simulink model "TECMD_Prototype"  (R2021a)
settings: Solver=daessc  StartTime=0.0  FixedStep=0.1  RelTol=1e-3  AbsTol=1e-3
libraries: nesl_utility x8, fl_lib x7, BatteryLibrary_lib x2
settings Model: Creator=widana_d  LastModifiedBy=widana_d
settings SolverCC: AutoScaleAbsTol=off  AlgebraicLoopSolver=TrustRegion
settings DataIOCC: SaveState=on
settings DebuggingCC: SymbolicDimsDataTypeCodeGenerationDiagnostic=none  SFMachineParentedDataDiag=warning
settings SFSimCC: CustomCodeUndefinedFunction=UseInterfaceOnly
settings SimscapeCC: SimscapeLogType=all  SimscapeLogSimulationStatistics=on  SimscapeLogDataHistory=10000

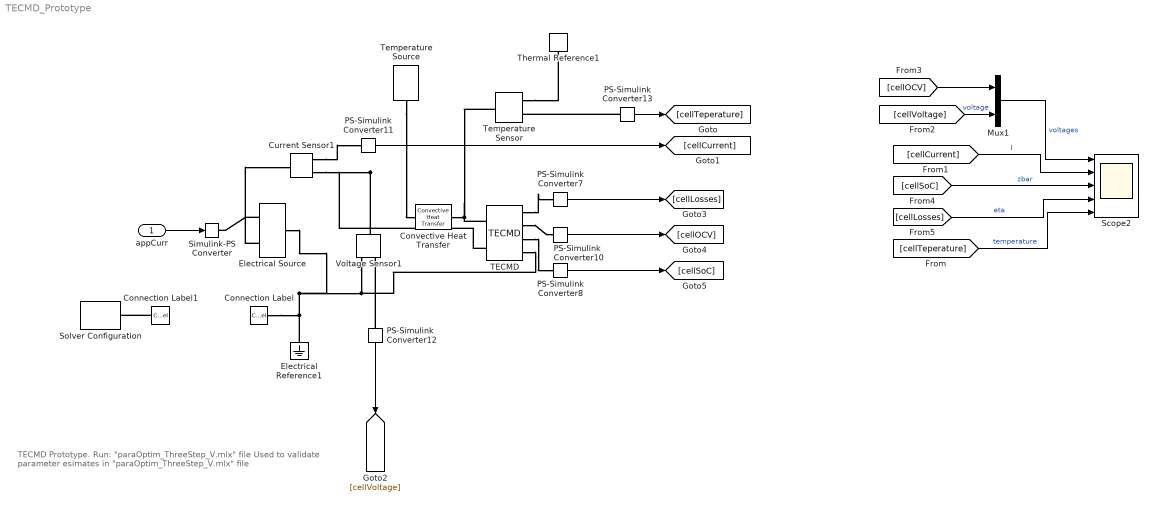
== system TECMD_Prototype ==
  note: TECMD Prototype.
      | Run: "paraOptim_ThreeStep_V.mlx" file
      | Used to validate parameter esimates in "paraOptim_ThreeStep_V.mlx" file
  appCurr : Inport
  Connection Label : ConnectionLabel  Label=solver
  Connection Label1 : ConnectionLabel  Label=solver
  Convective Heat Transfer : fl_lib/Thermal/Thermal Elements/Convective Heat Transfer  area=cellArea m^2  heat_tr_coeff=h W/(m^2 * K)  T_specify=off  T_priority=None  T=0 K  T_nominal_specify=off  T_nominal_unit=K  T_nominal_value=1  Q_specify=off  Q_priority=None  Q=0 W  Q_nominal_specify=off  Q_nominal_unit=W  Q_nominal_value=1
  Current Sensor1 : fl_lib/Electrical/Electrical Sensors/Current Sensor
  Electrical Reference1 : fl_lib/Electrical/Electrical Elements/Electrical Reference
  Electrical Source : BatteryLibrary_lib/Utilities/Electrical Source  inType=0
      settings: InternalSimscapePortConfiguration="{\"Bottom\":[{\"id\":\"n\",\"label\":\"-\",\"type\":\"foundation.electrical.electrical\"}],\"Left\":[{\"id\":\"inputSignal\",\"label\":\"Input\",\"type\":\"input\"}],\"Right\":[],\"Top\":[{\"id\":\"p\",\"label\":\"+\",\"type\":\"foundation.electrical.electrical\"}]}"
  Mux1 : Mux  Inputs=2
  PS-Simulink Converter{7..8,10..13} (6 alike) : nesl_utility/PS-Simulink Converter  PhysicalDomain=network_engine_domain  SubClassName=ps_output  LeftPortType=input  RightPortType=output  PseudoPeriodic=off  Frequencies=[]  Unit=inherit  AffineConversion=off
      settings: SourceProductName=Utilities
  Scope2 : Scope  NumInputPorts=5
  Simulink-PS Converter : nesl_utility/Simulink-PS Converter  PhysicalDomain=network_engine_domain  SubClassName=ps_input  LeftPortType=input  RightPortType=output  PseudoPeriodic=off  Frequencies=[]  NoiseDistribution=none  NoiseParameters=[]  Unit=1  AffineConversion=off  FilteringAndDerivatives=provide  SimscapeFilterOrder=1  InputFilterTimeConstant=0.001  UdotUserProvided=0
      settings: SourceProductBaseCode=PW,SS
  Solver Configuration : nesl_utility/Solver Configuration  PhysicalDomain=network_engine_domain  SubClassName=solver  LeftPortType=input  RightPortType=generic  Tones=[]  Harmonics=[]  SimulateNoise=off  Profile=off  UseLocalSampling=off  EnableSwitchedLinearOptims=on  FrequencyDomain=off  UseCCode=off  RelTol=0.001  AbsTol=1e-06  MinStep=1e-09  ToWorkspace=off  RevertToSquareIcSolve=off  NumHomotopyIterations=100  PhasorMode=off  PhasorModeNumHarmonics=1  DoDC=off  ResidualTolerance=1e-09  UseLocalSolver=off  LocalSolverChoice=NE_BACKWARD_EULER_ADVANCER  LocalSolverSampleTime=0.001  DoFixedCost=off  MaxNonlinIter=3  MaxModeIter=2  ComputeImpulses=off  ImpulseIterations=2  LinearAlgebra=auto  EquationFormulation=NE_TIME_EF  DelaysMemoryBudget=1024  AutomaticFiltering=on  FilteringTimeConstant=0.001  PartitionStorageMethod=AS_NEEDED  PartitionMemoryBudget=1024  PartitionMethod=ROBUST
      settings: SourceProductName=Utilities
  TECMD : BatteryLibrary_lib/Models/TECMD  RoRef=RoRef Ohm  RpRef=RpRef Ohm  TaupRef=TaupRef s  TauRef=TauRef s  Cn=Cn hr*A  z0=z0  Cp=Cp J/K  Tref=Tref K  Ea_Ro=Ea_Ro kJ/mol  Ea_Rp=Ea_Rp kJ/mol  Ea_Taup=Ea_Taup kJ/mol  Ea_Tau=Ea_Tau kJ/mol  T0=ambTemp K  refSoC=[0 : 100]' / 100  refOCV=[2.87226666666667, 2.96052812994699, 3.02804006137187, 3.09555199279676, 3.16306392422164, 3.2001291114499, 3.22684932876092, 3.25356954607195, 3.28028976338298, 3.30366251902926, 3.32391086783852, 3.34415921664777, 3.36440756545703, 3.38337736980428, 3.39585056120364, 3.40808169748128, 3.42031283375891, 3.43312236542483, 3.44403277212358, 3.45436831838031, 3.46470386463704, 3.47489460441589, 3.48578295282009, 3.49716895836194, 3.50855496390379, 3.51975057723135, 3.52990789728309, 3.54012269726924, 3.55033749725539, 3.56053403978798, 3.56876876393151, 3.57634734074831, 3.58392591756512, 3.59150449438192, 3.59837651292555, 3.60400711532064, 3.60963771771574, 3.61526832011083, 3.62087603938814, 3.62605990154572, 3.63124376370329, 3.63642762586086, 3.64172472997681, 3.64738310137943, 3.65304989960037, 3.6587166978213, 3.66472767182913, 3.67174598798367, 3.6788777371365, 3.68600948628932, 3.69349161904363, 3.7024953271603, 3.7118125338251, 3.7211297404899, 3.73077493215115, 3.74281715264455, 3.75539849306634, 3.76797983348813, 3.78054451462135, 3.79302677795269, 3.80637677297635, 3.81972676800001, 3.83307676302367, 3.84456984787373, 3.85430164068239, 3.86403343349106, 3.87376522629972, 3.88293282901064, 3.89107889951479, 3.89922497001894, 3.90737104052308, 3.91557874276785, 3.92399213081386, 3.93240787383325, 3.94082361685263, 3.94963150612215, 3.95966546646635, 3.96983594392408, 3.98000642138181, 3.99032598576655, 4.00126821478467, 4.01233626061718, 4.02340430644969, 4.03432201816434, 4.04382704177779, 4.05280216094291, 4.06177728010803, 4.07065703360974, 4.07626015949775, 4.08051431663774, 4.08476847377773, 4.08902263091772, 4.09345555380871, 4.09831742254355, 4.1031792912784, 4.10804116001324, 4.1155790937363, 4.12906316200268, 4.14254723026907, 4.15856111602972, 4.17532536875376]' V
      settings: InternalSimscapePortConfiguration="{\"Bottom\":[{\"id\":\"n\",\"label\":\"-\",\"type\":\"foundation.electrical.electrical\"}],\"Left\":[{\"id\":\"Hi\",\"label\":\"H\",\"type\":\"foundation.thermal.thermal\"}],\"Right\":[{\"id\":\"eta\",\"label\":\"Losses\",\"type\":\"output\"},{\"id\":\"OCV\",\"label\":\"OCV\",\"type\":\"output\"},{\"id\":\"zbar\",\"label\":\"SoC\",\"type\":\"output\"}],\"Top\":[{\"id\":\"p\",\"label\":\"+\",\"type\":\"foundation.electrical.electrical\"}]}"
  Temperature Sensor : fl_lib/Thermal/Thermal Sensors/Temperature Sensor
  Temperature Source : fl_lib/Thermal/Thermal Sources/Temperature Source  temperature=ambTemp K
  Thermal Reference1 : fl_lib/Thermal/Thermal Elements/Thermal Reference
  Voltage Sensor1 : fl_lib/Electrical/Electrical Sensors/Voltage Sensor
  wires:
  PS-Simulink Converter13/1 -> [cellTeperature]
  PS-Simulink Converter11/1 -> [cellCurrent]
  [cellOCV] -> Mux1/1
  [cellVoltage] -> Mux1/2  "voltage"
  Mux1/1 -> Scope2/1  "voltages"
  [cellCurrent] -> Scope2/2  "I"
  [cellTeperature] -> Scope2/5  "temperature"
  [cellSoC] -> Scope2/3  "zbar"
  [cellLosses] -> Scope2/4  "eta"
  PS-Simulink Converter12/1 -> [cellVoltage]
  appCurr/1 -> Simulink-PS Converter/1
  PS-Simulink Converter7/1 -> [cellLosses]
  PS-Simulink Converter10/1 -> [cellOCV]
  PS-Simulink Converter8/1 -> [cellSoC]
  connections:
  Electrical Reference1/LConn1 -- Electrical Source/RConn1 -- TECMD/RConn4 -- Voltage Sensor1/RConn2 -- Connection Label/LConn1
  Temperature Sensor/RConn1 -- Thermal Reference1/LConn1
  PS-Simulink Converter12/LConn1 -- Voltage Sensor1/RConn1
  PS-Simulink Converter13/LConn1 -- Temperature Sensor/RConn2
  Connection Label1/LConn1 -- Solver Configuration/RConn1
  Electrical Source/LConn1 -- Simulink-PS Converter/RConn1
  Voltage Sensor1/LConn1 -- TECMD/LConn2 -- Current Sensor1/RConn2
  TECMD/RConn1 -- PS-Simulink Converter7/LConn1
  TECMD/RConn2 -- PS-Simulink Converter10/LConn1
  TECMD/RConn3 -- PS-Simulink Converter8/LConn1
  Convective Heat Transfer/LConn1 -- TECMD/LConn1 -- Temperature Sensor/LConn1
  Temperature Source/LConn1 -- Convective Heat Transfer/RConn1
  Electrical Source/LConn2 -- Current Sensor1/LConn1
  Current Sensor1/RConn1 -- PS-Simulink Converter11/LConn1
